simulink model "copilot_closed_loop"  (R2026b)
settings: Solver=ode45  StopTime=simulationStopTime_demo  FixedStep=0.002  EnableMultiTasking=on
values from neighbouring files (symbols this model uses):
  Kp_demo = 2.25    [variables.mat]
settings Model: Creator=ecosgrov  LastModifiedBy=garellan
settings SolverCC: PositivePriorityOrder=on
settings DataIOCC: ReturnWorkspaceOutputs=off
settings DebuggingCC: ArithmeticOperatorsInVariantConditions=warning
settings SFSimCC: CustomCodeUndefinedFunction=UseInterfaceOnly  SimUseLocalCustomCode=off
settings RTWCC: RTWUseLocalCustomCode=off
settings CodeAppCC: StateflowObjectComments=on
settings ConfigComp: CovMetricSettings=ds

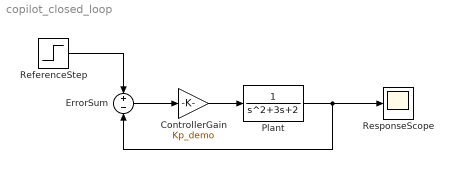
== system copilot_closed_loop ==
  ControllerGain : Gain  Gain=Kp_demo
  ErrorSum : Sum  Inputs=+-
  Plant : TransferFcn  Denominator=[1 3 2]
  ReferenceStep : Step  Time=0  FinalValue=stepAmplitude_demo  SampleTime=0
  ResponseScope : Scope
  wires:
  Plant/1 -> ResponseScope/1, ErrorSum/2
  ControllerGain/1 -> Plant/1
  ErrorSum/1 -> ControllerGain/1
  ReferenceStep/1 -> ErrorSum/1
